simulink model "Tp"  (R2017b)
settings: Solver=ode1  StartTime=0.0  StopTime=Inf  FixedStep=Te  RelTol=1e-3
PostLoadFcn:
  | , if any(exist('dsrtsu_mdlpostloadfcn', 'file') == [2, 3, 6]), try dsrtsu_mdlpostloadfcn('Execute', bdroot); catch fprintf('Error in PostLoadFcn (dsrtsu_mdlpostloadfcn) for model "%s":\n %s\n', bdroot, lasterr); end, end,
values from neighbouring files (symbols this model uses):
  largeurImpulsion = 50    [monCode.m]
  maPeriode = 8    [monCode.m]
  monAmplitude = 3.5    [monCode.m]
  monRetard = 1    [monCode.m]
  s0 = (p0d*p1d-DD)/(Kv_r*(1-DD))    [monCode.m]
  s1 = (1+DD-p0d-p1d)/(Kv_r*(1-DD))    [monCode.m]
  t0 = -(1-p1d)*p0d/(Kv*(1-DD))    [monCode.m]
  t1 = (1-p1d)/(Kv*(1-DD))    [monCode.m]
  Te = 0.001    [monCode.m]
libraries: rtilib1104 x2
Description:
  | Standard RTI1104 template.
  | Supported MATLAB version:  R2017b.
settings Model: Tag=RTI1104  DSRTSU_INTERNAL_RTI_VER=510  DSRTSU_INTERNAL_RTI_TYPE=rti1104  RTICANMMDATA=struct('GeneralSetupData',struct('modelroot','C:\Temp\UE520','generalsettings',struct('filesettings',struct('destfolder',struct('Name','RTICANMM_FILES','Check',1),'buildfolder',struct('Name','.','Check',1),'AbsDestfolder',struct('Name','C:\Temp\UE520\RTICANMM_FILES'),'AbsBuildfolder',struct('Name','C:\Temp\UE520'))),'options',struct('addpaths',1,'rmpaths',1,'addtrcexclusion',logical(1),'cannavigator',struct('checkmonitoring',0),'show_usrtrc',0,'use_usrtrc',0),'advanced',struct('options',[1 1 1 1 1 1 1 1 1 1 1 1 1 1 1 1 1 1 1 1 1 1 1 1 1 1 1 1 1 1 1 1 1 1 1 1 1 1 1 1 1 1 1 1 1 1 1 1 1 1 1 1 1 1 1 1 1 1 1 1 1 1 1 1 1 1 1 1 1 1 1 1 1 1 1 1 1 1 1 1 1 1 1 1 1 1 1 1 1 1 1 1 1 1 1 1 1 1 1 1]),'MPSetup',{{}},'modelname','Tp','block','Tp'))  DSRTSU_INTERNAL_RTIFLEXRAYCONFIG=110  DSRTSU_INTERNAL_RTIFPGA=110  Creator=gbouchy  LastModifiedBy=gbouchy
settings OptimizationCC: BlockReduction=off  OptimizeBlockIOStorage=off  BufferReuse=off  GlobalBufferReuse=off  ExpressionFolding=off  LocalBlockOutputs=off
settings HardwareCC: ProdBitPerPointer=32  ProdBitPerSizeT=32  ProdBitPerPtrDiffT=32  ProdLargestAtomicInteger=Integer  ProdEndianess=BigEndian  ProdWordSize=32  ProdHWDeviceType=Custom Processor->Custom  TargetIntDivRoundTo=Zero  TargetEndianess=BigEndian  TargetHWDeviceType=Custom Processor->Custom
settings SFSimCC: MATLABDynamicMemAlloc=off
settings RTWCC: SystemTargetFile=rti1104.tlc  MakeCommand=make_rti  TemplateMakefile=rti1104.tmf  Description=dSPACE DS1104 Hardware Platform
settings CodeAppCC: StateflowObjectComments=on
settings STFCustomTargetCC: ParMdlRefBuildCompliant=on  GRTInterface=off  SystemTargetFile=rti1104.tlc
settings GRTTargetCC: TargetLangStandard=C89/C90 (ANSI)  CompOptLevelCompliant=off  ConcurrentExecutionCompliant=off  CombineOutputUpdateFcns=off  MatFileLogging=off  CPPClassGenCompliant=off  UseToolchainInfoCompliant=off
settings ConfigComp: CovMetricSettings=dswe

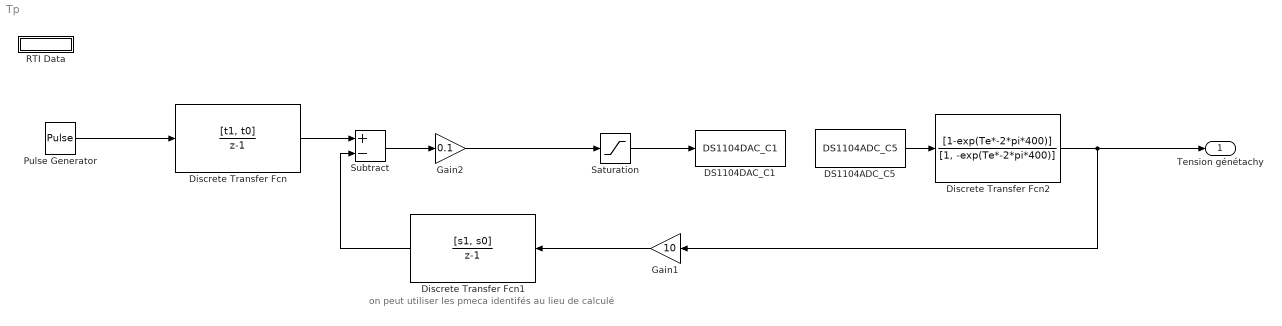
== system Tp ==
  note: on peut utiliser les pmeca identifés au lieu de calculé
  DS1104ADC_C5 : rtilib1104/DS1104 MASTER PPC/DS1104ADC_C5  ChannelNo=5  TriggerMode=0  Reserved1=[]  Reserved2=[]  Reserved3=[]  Reserved4=[]  DialogFcn=gui1104adc  UnitName={ 'DS1104ADC_C' }  UnitValues={ 5 }  DSProperties=struct('RTI',struct('Version',uint32(1),'BlockType',struct('isSLSource',uint8(1),'isSLSink',uint8(0),'isHWSource',uint8(1),'isHWSink',uint8(0),'isSetup',uint8(0),'isInline',uint8(1),'isNonInline',uint8(0),'isInterrupt',uint8(0),'isChannelwise',uint8(1)),'IOBoardType','DS1104MASTER','UnitType','ADC','Identifier','ADC','DialogType','ML','BlockSet','NONE','SlaveProcessor','NONE'))
      settings: SourceProductName=dSPACE RTI1104
  DS1104DAC_C1 : rtilib1104/DS1104 MASTER PPC/DS1104DAC_C1  ChannelNo=1  InitValue=0  TermMode=1  TermValue=0  Reserved1=[]  Reserved2=[]  Reserved3=[]  Reserved4=[]  DialogFcn=gui1104dac  UnitName={ 'DS1104DAC_C'}  UnitValues={ 1 }  DSProperties=struct('RTI',struct('Version',uint32(1),'BlockType',struct('isSLSource',uint8(0),'isSLSink',uint8(1),'isHWSource',uint8(0),'isHWSink',uint8(1),'isSetup',uint8(0),'isInline',uint8(1),'isNonInline',uint8(0),'isInterrupt',uint8(0),'isChannelwise',uint8(1)),'IOBoardType','DS1104MASTER','UnitType','DAC','Identifier','DAC','DialogType','ML','BlockSet','NONE','SlaveProcessor','NONE'))
      settings: SourceProductName=dSPACE RTI1104
  Discrete Transfer Fcn : DiscreteTransferFcn  Numerator=[t1, t0]  Denominator=[1 -1]
  Discrete Transfer Fcn1 : DiscreteTransferFcn  Numerator=[s1, s0]  Denominator=[1 -1]
  Discrete Transfer Fcn2 : DiscreteTransferFcn  Numerator=[1-exp(Te*-2*pi*400)]  Denominator=[1, -exp(Te*-2*pi*400)]
  Gain1 : Gain  Gain=10
  Gain2 : Gain  Gain=0.1
  Pulse Generator : DiscretePulseGenerator  PulseType=Time based  Amplitude=monAmplitude  Period=maPeriode  PulseWidth=largeurImpulsion  PhaseDelay=monRetard
  RTI Data : Subsystem  Tag=struct('RTIDataServer',struct('RTIDataServerVs','2','RTIModelDescription','struct(''main'',''Tp'',''sub'','''',''isMp'',0)'))  LoadFcn="if exist('rtidc'), try,  rtidc('DataHostBlockClbLoad', gcbh); catch, disp(['Warning: ''LoadFcn'' for RTI Data block failed: ' lasterr]); end, end,"  mask(RTI_DATA_HOST){}
      mask help:
      | RTI Data Block.
      | This block is used by RTI to store internal model-dependent data.
      | Please keep this block on the root level of the model. Deleting this block will result in data loss.
      |
      | NEVER DELETE OR COPY THIS BLOCK!
      settings: CopyFcn="if exist('rtidc'), try,  rtidc('DataHostBlockClbCopy', gcbh); catch, disp(['Warning: ''CopyFcn'' for RTI Data block failed: ' lasterr]); end, end,"  DeleteFcn="if exist('rtidc'), try,  rtidc('DataHostBlockClbDelete', gcbh); catch, disp(['Warning: ''DeleteFcn'' for RTI Data block failed: ' lasterr]); end, end,"  ModelCloseFcn="if exist('rtidc'), try,  rtidc('DataHostBlockClbModelClose', gcbh); catch, disp(['Warning: ''ModelCloseFcn'' for RTI Data block failed: ' lasterr]); end, end,"  PreSaveFcn="if exist('rtidc'), try,  rtidc('DataHostBlockClbPreSave', gcbh); catch, disp(['Warning: ''PreSaveFcn'' for RTI Data block failed: ' lasterr]); end, end,"  PostSaveFcn="if exist('rtidc'), try,  rtidc('DataHostBlockClbPostSave', gcbh); catch, disp(['Warning: ''PostSaveFcn'' for RTI Data block failed: ' lasterr]); end, end,"  NameChangeFcn="if exist('rtidc'), try,  rtidc('DataHostBlockClbNameChange', gcbh); catch, disp(['Warning: ''NameChangeFcn'' for RTI Data block failed: ' lasterr]); end, end,"
      mask Help:
      | RTI Data Block.
      | This block is used by RTI to store internal model-dependent data.
      | Please keep this block on the root level of the model. Deleting this block will result in data loss.
      | 
      | NEVER DELETE OR COPY THIS BLOCK!
      mask Display:
      | text(0.5, 0.5, 'RTI Data', 'HorizontalAlignment', 'center');
      | plot([1 0]);
  Saturation : Saturate  UpperLimit=1  LowerLimit=-1
  Subtract : Sum  Inputs=+-
  "Tension génétachy " : Outport
  wires:
  DS1104ADC_C5/1 -> Discrete Transfer Fcn2/1
  Saturation/1 -> DS1104DAC_C1/1
  Pulse Generator/1 -> Discrete Transfer Fcn/1
  Discrete Transfer Fcn/1 -> Subtract/1
  Subtract/1 -> Gain2/1
  Discrete Transfer Fcn1/1 -> Subtract/2
  Gain1/1 -> Discrete Transfer Fcn1/1
  Gain2/1 -> Saturation/1
  Discrete Transfer Fcn2/1 -> Gain1/1, "Tension génétachy "/1

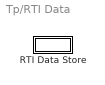
== system Tp/RTI Data ==
  RTI Data Store : Subsystem  Tag="struct('private',struct('version',struct('dsVer',uint32(2),'dsVerCreation',uint32(2),'RTI',struct('ver','7.9','type','RTI1104')),'access',struct('type','Model','isPerm',1,'created',['07-Feb-2023 14:37:24'],'modified',['14-Feb-2023 17:57:38'],'location','')),'public',struct('main',struct('data',[]),'sub',struct('name',{{'Tp'}},'data',{{struct('TH',struct('thTaskInfo',struct('taskType',{'TIMER','HWINT','TMRINT','SWINT','GLINT'},'tasksNumOf',{1,0,0,0,0},'srcIds',{{'TIMERA'},{},{},{},{}},'taskNames',{{['Timer Task 1']},{},{},{},{}})),'th_tc',struct('dataType','TASK','taskGroupId','','taskGroupList',{{}},'taskSchedulingPolicy','FCFS','taskType','TIMER','blkh',-1,'srcId','TIMERA','srcSgnName',['Timer A interrupt'],'srcCpuName','','taskName',['Timer Task 1  [0.001] s'],'taskNameDisplayExt','','smplTime',0.001,'smplTimeOffs',0,'hasFixedPriority',0,'priority',1,'hasFixedOvc',0,'ovcType',1,'ovcMax',1),'tc_th',struct('dataType','TASK','taskGroupId','','taskGroupList',{{}},'taskSchedulingPolicy','FCFS','taskType','TIMER','blkh',-1,'srcId','TIMERA','srcSgnName',['Timer A interrupt'],'srcCpuName','','taskName',['Timer Task 1  [0.001] s'],'taskNameDisplayExt','','smplTime',0.001,'smplTimeOffs',0,'hasFixedPriority',0,'priority',1,'hasFixedOvc',0,'ovcType',1,'ovcMax',1))}})))"  mask(RTI_DATA_STORE){}
      mask help:
      | RTI Data Store Block. This block is used by RTI to store internal model dependent data. Deleting this block will result in data loss.
      |
      | NEVER DELETE, COPY, OR MODIFY THIS BLOCK!
      mask Help:
      | RTI Data Store Block. This block is used by RTI to store internal model dependent data. Deleting this block will result in data loss.
      | 
      | NEVER DELETE, COPY, OR MODIFY THIS BLOCK!
      mask Display: text(0.5, 0.5, ' ', 'HorizontalAlignment', 'center');

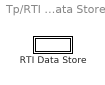
== system Tp/RTI Data/RTI Data Store ==
  RTI Data Store : Subsystem  mask(RTI_DATA_STORE){}
      mask help:
      | RTI Data Store Block. This block is used by RTI to store internal model dependent data. Deleting this block will result in data loss.
      |
      | NEVER DELETE, COPY, OR MODIFY THIS BLOCK!
      mask Help:
      | RTI Data Store Block. This block is used by RTI to store internal model dependent data. Deleting this block will result in data loss.
      | 
      | NEVER DELETE, COPY, OR MODIFY THIS BLOCK!
      mask Display: text(0.5, 0.5, ' ', 'HorizontalAlignment', 'center');

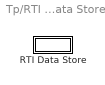
== system Tp/RTI Data/RTI Data Store/RTI Data Store ==
  RTI Data Store : Subsystem  mask(RTI_DATA_STORE){}
      mask help:
      | RTI Data Store Block. This block is used by RTI to store internal model dependent data. Deleting this block will result in data loss.
      |
      | NEVER DELETE, COPY, OR MODIFY THIS BLOCK!
      mask Help:
      | RTI Data Store Block. This block is used by RTI to store internal model dependent data. Deleting this block will result in data loss.
      | 
      | NEVER DELETE, COPY, OR MODIFY THIS BLOCK!
      mask Display: text(0.5, 0.5, ' ', 'HorizontalAlignment', 'center');

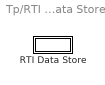
== system Tp/RTI Data/RTI Data Store/RTI Data Store/RTI Data Store ==
  RTI Data Store : Subsystem  mask(RTI_DATA_STORE){}
      mask help:
      | RTI Data Store Block. This block is used by RTI to store internal model dependent data. Deleting this block will result in data loss.
      |
      | NEVER DELETE, COPY, OR MODIFY THIS BLOCK!
      mask Help:
      | RTI Data Store Block. This block is used by RTI to store internal model dependent data. Deleting this block will result in data loss.
      | 
      | NEVER DELETE, COPY, OR MODIFY THIS BLOCK!
      mask Display: text(0.5, 0.5, ' ', 'HorizontalAlignment', 'center');

== system Tp/RTI Data/RTI Data Store/RTI Data Store/RTI Data Store/RTI Data Store ==
